simulink model "uacs_aero_test"  (R2024a)
settings: Solver=ode4  StartTime=0.0  StopTime=sim_t_end  FixedStep=sim_ts_ctrl  RelTol=1e-3
PreLoadFcn:
  | p=fileparts(fileparts(get_param(bdroot,'FileName')));addpath(p,fullfile(p,'params'),fullfile(p,'plant'),fullfile(p,'control'),fullfile(p,'sim'),fullfile(p,'run'),fullfile(p,'verify'),'-begin');uacs_go
InitFcn:
  | p=fileparts(fileparts(get_param(bdroot,'FileName')));addpath(p,fullfile(p,'params'),fullfile(p,'plant'),fullfile(p,'control'),fullfile(p,'sim'),fullfile(p,'run'),fullfile(p,'verify'),'-begin');uacs_ensure
undefined symbols (not defined in the file): sim_c_one
libraries: simulink x7
settings Model: Creator=Ash Trailer  LastModifiedBy=Ash Trailer
settings DataIOCC: SaveFormat=StructureWithTime
settings DebuggingCC: AlgebraicLoopMsg=error

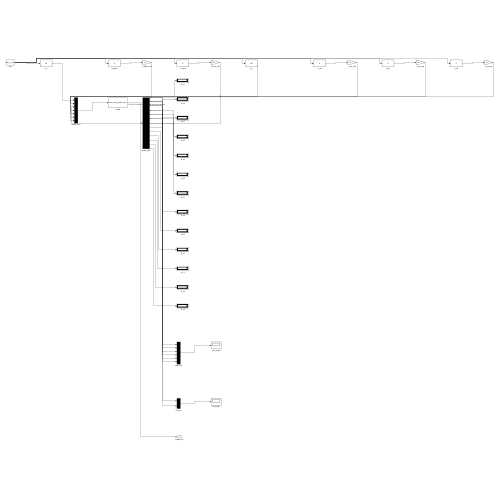
[thumbnail: Simulink's stored preview of the top-level diagram]
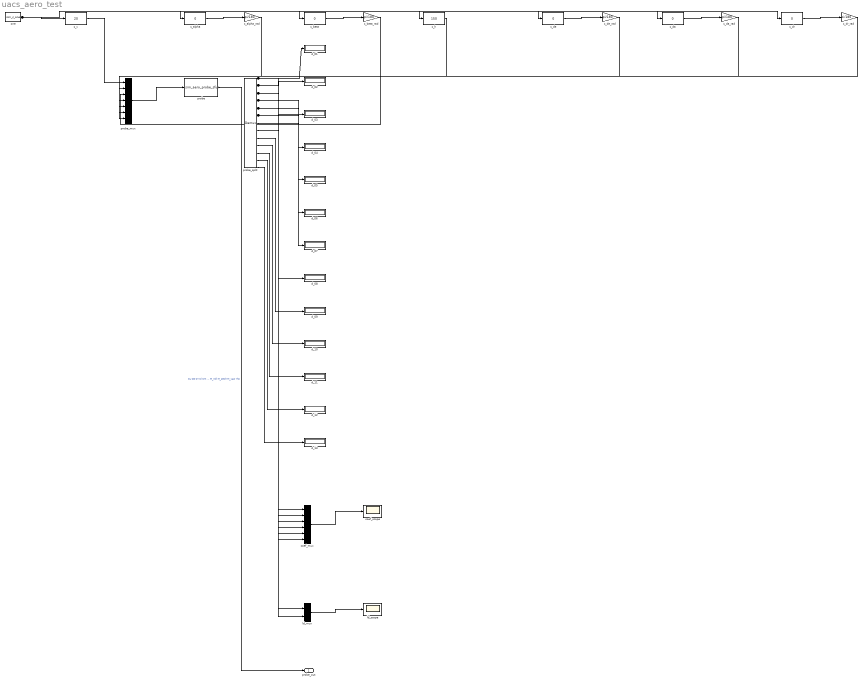
== system uacs_aero_test ==
  coef_mux : Mux  Inputs=6
  coef_scope : Scope
  d_01 : Display
  d_02 : Display
  d_03 : Display
  d_04 : Display
  d_05 : Display
  d_06 : Display
  d_07 : Display
  d_08 : Display
  d_09 : Display
  d_{10..13} (4 alike) : Display
  ld_mux : Mux  Inputs=2
  ld_scope : Scope
  one : Constant  Value=sim_c_one
  probe : M-S-Function  FunctionName=sim_aero_probe_sfun
  probe_mux : Mux  Inputs=7
  probe_split : Demux  Outputs=13
  s_alpha : simulink/Math Operations/Slider Gain  gain=0  low=-5  high=20
  s_alpha_rad : Gain  Gain=pi/180
  s_beta : simulink/Math Operations/Slider Gain  gain=0  low=-15  high=15
  s_beta_rad : Gain  Gain=pi/180
  s_da : simulink/Math Operations/Slider Gain  gain=0  low=-25  high=25
  s_da_rad : Gain  Gain=pi/180
  s_de : simulink/Math Operations/Slider Gain  gain=0  low=-25  high=25
  s_de_rad : Gain  Gain=pi/180
  s_dr : simulink/Math Operations/Slider Gain  gain=0  low=-25  high=25
  s_dr_rad : Gain  Gain=pi/180
  s_h : simulink/Math Operations/Slider Gain  gain=150  low=0  high=400
  s_v : simulink/Math Operations/Slider Gain  gain=20  low=5  high=35
  probe_out : Outport
  wires:
  one/1 -> s_v/1, s_alpha/1, s_beta/1, s_h/1, s_de/1, s_da/1, s_dr/1
  s_alpha/1 -> s_alpha_rad/1
  s_beta/1 -> s_beta_rad/1
  s_de/1 -> s_de_rad/1
  s_da/1 -> s_da_rad/1
  s_dr/1 -> s_dr_rad/1
  s_v/1 -> probe_mux/1
  s_alpha_rad/1 -> probe_mux/2
  s_beta_rad/1 -> probe_mux/3
  s_h/1 -> probe_mux/4
  s_de_rad/1 -> probe_mux/5
  s_da_rad/1 -> probe_mux/6
  s_dr_rad/1 -> probe_mux/7
  probe_mux/1 -> probe/1
  probe_split/1 -> d_01/1, coef_mux/1, ld_mux/1
  probe_split/2 -> d_02/1, coef_mux/2, ld_mux/2
  probe_split/3 -> d_03/1, coef_mux/3
  probe_split/4 -> d_04/1, coef_mux/4
  probe_split/5 -> d_05/1, coef_mux/5
  probe_split/6 -> d_06/1, coef_mux/6
  probe_split/7 -> d_07/1
  probe_split/8 -> d_08/1
  probe_split/9 -> d_09/1
  probe_split/10 -> d_10/1
  probe_split/11 -> d_11/1
  probe_split/12 -> d_12/1
  probe_split/13 -> d_13/1
  coef_mux/1 -> coef_scope/1
  ld_mux/1 -> ld_scope/1
  probe/1 -> probe_out/1  "CL CD CY Cl Cm Cn L D Y M_roll M_pitch M_yaw rho"
